simulink model "MMC_phase_hackathon_consensus_PWM_JABBAR_20260927"  (R2024b)
settings: Solver=FixedStepDiscrete  StartTime=t_init_sim  StopTime=sim_time  FixedStep=Ts  RelTol=1e-3
values from neighbouring files (symbols this model uses):
  a = 1    [script_MMC_phase_hackathon_consensus_PWM_JABBAR_20260927.m]
  C1low1_active = 1    [script_MMC_phase_hackathon_consensus_PWM_JABBAR_20260927.m]
  C2low1_active = 1    [script_MMC_phase_hackathon_consensus_PWM_JABBAR_20260927.m]
  C_bus = 4400e-6    (= 0.0044)    [script_MMC_phase_hackathon_consensus_PWM_JABBAR_20260927.m]
  C_M_extra = C_m-twist_high_side_C    [script_MMC_phase_hackathon_consensus_PWM_JABBAR_20260927.m]
  f0 = 50    [script_MMC_phase_hackathon_consensus_PWM_JABBAR_20260927.m]
  feeder_current_lower_rate_limit = -10    [script_MMC_phase_hackathon_consensus_PWM_JABBAR_20260927.m]    (also in twist_parameters.m = -500)
  feeder_current_tab = [0.328 0.217 0.162 0.132 0.109 0.094 0.083 0.075 0.068 0.062 0.058 0.054 ... (42 elements, 14x3)]    [feeder_current.mat]
  feeder_current_upper_rate_limit = 0.386/(20e-3)    (= 19.3)    [twist_parameters.m]
  is6VExternallySupplied = true    [script_MMC_phase_hackathon_consensus_PWM_JABBAR_20260927.m]
  isFeederJumperOpen = true    [script_MMC_phase_hackathon_consensus_PWM_JABBAR_20260927.m]
  L_arm = 100e-3    (= 0.1)    [script_MMC_phase_hackathon_consensus_PWM_JABBAR_20260927.m]
  m = 1    [script_MMC_phase_hackathon_consensus_PWM_JABBAR_20260927.m]
  power_losses = false    [script_MMC_phase_hackathon_consensus_PWM_JABBAR_20260927.m]
  R = 30    [script_MMC_phase_hackathon_consensus_PWM_JABBAR_20260927.m]
  R_arm = 0.2    [script_MMC_phase_hackathon_consensus_PWM_JABBAR_20260927.m]
  source_V = 0    [script_MMC_phase_hackathon_consensus_PWM_JABBAR_20260927.m]
  time_charge = 0.1    [script_MMC_phase_hackathon_consensus_PWM_JABBAR_20260927.m]
  time_decharge = 1.5    [script_MMC_phase_hackathon_consensus_PWM_JABBAR_20260927.m]
  Ts = 5e-7    (= 5e-07)    [script_MMC_phase_hackathon_consensus_PWM_JABBAR_20260927.m]
  twist_data_acquisition_delay = 50e-9    (= 5e-08)    [script_MMC_phase_hackathon_consensus_PWM_JABBAR_20260927.m]    (also in twist_parameters.m)
  twist_data_sampling_period = 1/twist_freq_data_sampling    (= 5e-05)    [script_MMC_phase_hackathon_consensus_PWM_JABBAR_20260927.m]    (also in twist_parameters.m)
  twist_dead_time = 200e-9    (= 2e-07)    [twist_parameters.m]
  twist_freq_switching = 200e3    (= 200000)    [twist_parameters.m]
  twist_high_side_adc_R = 1/(1/2e6 + 1/2e6 + 1/(330e3+5.6e3))    (= 251272.836178)    [twist_parameters.m]
  twist_high_side_C = 33e-6*4 + 4.7e-6*12    (= 0.0001884)    [twist_parameters.m]
  twist_high_side_feeder_R = 47e3+4.7e3    (= 51700)    [twist_parameters.m]
  twist_high_side_rC = 0.1    [twist_parameters.m]
  twist_low_side_adc_R = 150e3+470    (= 150470)    [twist_parameters.m]
  twist_low_side_C_ceramic = 3*4.7e-6    (= 1.41e-05)    [twist_parameters.m]
  twist_low_side_C_electrolytic = 47e-6    (= 4.7e-05)    [twist_parameters.m]
  twist_low_side_L = 33e-6    (= 3.3e-05)    [twist_parameters.m]
  twist_low_side_rC = 700e-3    (= 0.7)    [twist_parameters.m]
  twist_low_side_rL = 20e-3    (= 0.02)    [twist_parameters.m]
  twist_R_VCC = (tau_VCC/twist_high_side_C  - twist_high_side_rC)/(1-(tau_VCC/twist_high_side_C - twist_high_side_rC)/R_parallel)    (= 1110.74997822)    [twist_parameters.m]
  VDC = 48    [script_MMC_phase_hackathon_consensus_PWM_JABBAR_20260927.m]
undefined symbols (not defined in the file or in its folder): C_SM, feeder_current, gcbh, sps_rtmsupport, twist_low_side_lC
libraries: spsSeriesRLCBranchLib x135, spsTriangleGeneratorLib x60, spsMosfetLib x60, spsCurrentMeasurementLib x43, spsVoltageMeasurementLib x35, spsControlledCurrentSourceLib x30, spsDiodeLib x22, spsIdealSwitchLib x20, spsControlledVoltageSourceLib x1, spsGroundLib x1, spspowerguiLib x1
(part 8 of 19)

== system MMC_phase_hackathon_consensus_PWM_JABBAR_20260927/ /Subsystem/Subsystem1/Hardware M3/Feeder block ==
  note: Note:
      | Feeder chracteristics changed to consider threshold voltages (Vth_start = 9.7 V and Vth_stop = 8.9 V).
      | -When started, its VIN PIN consums the current generated by the lookup table fed with consumption experimental data from OwnTech.
      | -When stopped, its VIN PIN no longer consums current but its VCC PIN is modelled as a resistance calculated to match experimental results.
      | -When externally supply the 6 V used by the board, the feeder consums a constant 11.2 mA current when above threshold voltage, which is its correspondent to the minimum current in datasheet (15 mA).
  duty_cycle : Inport
  vHMeas : Inport  Port=2
  2-D Lookup Table : Lookup_n-D  Commented=on  LookupTableObject=feeder_current_tab  BreakpointsSpecification=Even spacing  BreakpointsForDimension1=[1:4]  BreakpointsForDimension2=[1:3]  BreakpointsForDimension1FirstPoint=feeder_VHigh_min  BreakpointsForDimension2FirstPoint=feeder_duty_min  BreakpointsForDimension1Spacing=feeder_VHigh_spacing  BreakpointsForDimension2Spacing=feeder_duty_spacing  TableSource=Input port  Table=feeder_current  InternalRulePriority=Speed  RndMeth=Simplest
      settings: InputPortMap=u0,u1,p221
  Constant11 : Constant  Commented=on  Value=is6VExternallySupplied
  Constant12 : Constant  Commented=on  Value=isFeederJumperOpen
  Constant2 : Constant  Commented=on  Value=0
  Constant4 : Constant  Commented=on  Value=0
  Constant5 : Constant  Commented=on
  Constant6 : Constant  Commented=on  Value=0
  Constant7 : Constant  Commented=on  Value=feeder_current_tab
  GreaterThan : RelationalOperator  Commented=on  Operator=>  OutDataTypeStr=boolean  RndMeth=Simplest  InputSameDT=off
  MATLAB Function : MATLAB Function  Commented=on  TreatAsAtomicUnit=on
  Memory : Memory  Commented=on  InheritSampleTime=on  LinearizeAsDelay=on
  Rate Limiter : RateLimiter  Commented=on  RisingSlewLimit=feeder_current_upper_rate_limit  FallingSlewLimit=feeder_current_lower_rate_limit  SampleTimeMode=inherited
  Switch : Switch  Commented=on  Criteria=u2 > Threshold  Threshold=2.05  SaturateOnIntegerOverflow=off  InputSameDT=off
  Switch10 : Switch  Commented=on  Criteria=u2 > Threshold  SaturateOnIntegerOverflow=off  InputSameDT=off
  Switch11 : Switch  Commented=on  Criteria=u2 > Threshold  SaturateOnIntegerOverflow=off  InputSameDT=off
  Switch9 : Switch  Commented=on  Criteria=u2 > Threshold  SaturateOnIntegerOverflow=off  InputSameDT=off
  Qjumper : Outport
  feeder_current : Outport  Port=2
  QVCC : Outport  Port=3
  wires:
  GreaterThan/1 -> Memory/1
  Constant2/1 -> GreaterThan/2
  Constant5/1 -> Switch11/3
  MATLAB Function/1(y) -> GreaterThan/1, Rate Limiter/1
  Constant4/1 -> Switch/3
  Switch/1 -> QVCC/1
  Switch10/1 -> Switch/1
  Memory/1 -> MATLAB Function/4(active_1)
  Constant6/1 -> Switch11/1, Switch10/1, Switch9/1
  Constant12/1 -> Switch11/2, Switch9/2, Switch10/2
  Constant11/1 -> MATLAB Function/3(isfeederdisabled)
  2-D Lookup Table/1 -> MATLAB Function/1(i_feeder)
  Rate Limiter/1 -> Switch9/3
  MATLAB Function/2(Q_VCC) -> Switch10/3
  Switch9/1 -> feeder_current/1
  Constant7/1 -> 2-D Lookup Table/3
  duty_cycle/1 -> 2-D Lookup Table/2
  vHMeas/1 -> MATLAB Function/2(vC), Switch/2, 2-D Lookup Table/1
  Switch11/1 -> Qjumper/1

== system MMC_phase_hackathon_consensus_PWM_JABBAR_20260927/ /Subsystem/Subsystem1/Hardware M3/HRTimA_1 ==
  note: PWM Timer Model
  note: Note 2:
      | All sampling times inferior than Ts = 1e-6 were desactivated or changed to Ts to reduce simulation duration
  note: Note 3:
      | PWM generator original resolution value at 100 ns
  note: Note 1:
      | HRTim modified adding block mode, equivalent to shield.power.stop(ALL);
  Duty cycle input : Inport
  Block : Inport  Port=2
  Constant : Constant  Value=0
  Dead Time : TransportDelay  Commented=on  DelayTime=twist_dead_time
  Demux : Demux  Outputs=2
  Logical Operator : Logic  AllPortsSameDT=off  OutDataTypeStr=boolean
  PWM Generator (2-Level) : Subsystem  AncestorBlock=|  DialogController=POWERSYS.PowerSysDialog  LoadFcn=sps_rtmsupport('LoadFcn', gcbh);  StartFcn=sps_rtmsupport('StartFcn', gcbh);  StopFcn=sps_rtmsupport('StopFcn', gcbh);  BlockChoice=InternalUref  mask(PWM Generator (2-Level)){ModulatorType=Single-phase half-bridge (2 pulses), ModulatorMode=Unsynchronized, Fc=twist_freq_switching, Pc=144, nF=27, MinMax=[0 1], SamplingTechnique=Symmetrical regular (single edge), ModulatingSignals=off, m=0.8, Freq=60, Phase=0, Ts=Ts, ShowCarrierOutport=off}
      | spsPWMGenerator2LevelLib/PWM Generator
      | (2-Level)
      mask prompts: ModulatorType "Generator type:"; ModulatorMode "Mode of operation:"; Fc "Frequency (Hz):"; Pc "Initial phase (degrees):"; nF "Switching ratio (carrier frequency / output frequency):"; MinMax "Minimum and maximum values: [ Min  Max ]"; SamplingTechnique "Sampling technique:"; ModulatingSignals "Internal generation of reference signal"; m "Modulation index:"; Freq "Frequency (Hz):"; Phase "Phase (degrees):"; Ts "Sample time (s):"; ShowCarrierOutport "Show measurement port"
      mask help:
      | Generate pulses for PWM-controlled 2-Level converter, using carrier-based two-level PWM method. The block can control switching devices of single-phase half-bridge, single-phase full-bridge (unipolar or bipolar modulation) or three-phase bridge.
      |
      | When the Synchronized mode of operation is selected, a second input is added to the block, and the internal generation of modulating signal is disabled. Use input 2 (wt) to synchronize the carrier.
      mask init:
      | sps = powericon('PWMGenerator2LevelInit',gcb,ModulatorType,SamplingTechnique,ModulatorMode,nF,Fc,MinMax,Pc,ShowCarrierOutport,ModulatingSignals,m,Freq,Phase,Ts);
      settings: CopyFcn=sps_rtmsupport('CopyFcn', gcbh);  DeleteFcn=sps_rtmsupport('DeleteFcn', gcbh);  UndoDeleteFcn=sps_rtmsupport('UndoDeleteFcn', gcbh);  ModelCloseFcn=sps_rtmsupport('ModelCloseFcn', gcbh);  PreSaveFcn=sps_rtmsupport('PreSaveFcn', gcbh);  PostSaveFcn=sps_rtmsupport('PostSaveFcn', gcbh);  NameChangeFcn=sps_rtmsupport('NameChangeFcn', gcbh);  PreCopyFcn=sps_rtmsupport('PreCopyFcn', gcbh);  OpenFcn="sps_rtmsupport('OpenFcn', gcbh, [1   2   7   8  13]);"  CloseFcn=sps_rtmsupport('CloseFcn', gcbh);  PreDeleteFcn=sps_rtmsupport('PreDeleteFcn', gcbh);
      mask Help: helpview(psbhelp);
      mask TypeOptions ModulatorType: Single-phase half-bridge (2 pulses) | Single-phase full-bridge (4 pulses) | Single-phase full-bridge - Bipolar modulation (4 pulses) | Three-phase bridge (6 pulses)
      mask TypeOptions ModulatorMode: Synchronized | Unsynchronized
      mask Callback ModulatorMode: powericon('PWMGenerator2LevelCback',gcb);
      mask TypeOptions SamplingTechnique: Natural | Asymmetrical regular (double edge) | Symmetrical regular (single edge)
      mask Callback ModulatingSignals: powericon('PWMGenerator2LevelCback',gcb);
      mask DialogControl Container3 Prompt: Carrier
      mask DialogControl ModulatingSignalParameters Prompt: Reference signal
  Peak acq : ZeroOrderHold  Commented=on  SampleTime=twist_data_acquisition_delay
  Switch : Switch  Criteria=u2 > Threshold  SaturateOnIntegerOverflow=off  InputSameDT=off
  Switch1 : Switch  Criteria=u2 > Threshold  SaturateOnIntegerOverflow=off  InputSameDT=off
  High-Side Q : Outport
  Low-Side Q : Outport  Port=2
  Carry Leg : Outport  Port=3
  wires:
  Demux/1 -> Switch/3  "high side"
  Duty cycle input/1 -> PWM Generator (2-Level)/1(Uref)  "duty_cycle"
  PWM Generator (2-Level)/2(Carry) -> Carry Leg/1, Peak acq/1  "carrier"
  Block/1 -> Switch/2, Switch1/2  "block"
  Demux/2 -> Switch1/3  "low side"
  Switch1/1 -> Low-Side Q/1
  Switch/1 -> High-Side Q/1
  Constant/1 -> Switch1/1, Switch/1
  PWM Generator (2-Level)/1(P) -> Demux/1, Dead Time/1, Logical Operator/1, Logical Operator/2  "PWM_out"

== system MMC_phase_hackathon_consensus_PWM_JABBAR_20260927/ /Subsystem/Subsystem1/Hardware M3/HRTimA_2 ==
  note: PWM Timer Model
  note: Note 2:
      | All sampling times inferior than Ts = 1e-6 were desactivated or changed to Ts to reduce simulation duration
  note: Note 3:
      | PWM generator original resolution value at 100 ns
  note: Note 1:
      | HRTim modified adding block mode, equivalent to shield.power.stop(ALL);
  Duty cycle input : Inport
  Block : Inport  Port=2
  Constant : Constant  Value=0
  Dead Time : TransportDelay  Commented=on  DelayTime=twist_dead_time
  Demux : Demux  Outputs=2
  Logical Operator : Logic  AllPortsSameDT=off  OutDataTypeStr=boolean
  PWM Generator (2-Level) : Subsystem  AncestorBlock=|  DialogController=POWERSYS.PowerSysDialog  LoadFcn=sps_rtmsupport('LoadFcn', gcbh);  StartFcn=sps_rtmsupport('StartFcn', gcbh);  StopFcn=sps_rtmsupport('StopFcn', gcbh);  BlockChoice=InternalUref  mask(PWM Generator (2-Level)){ModulatorType=Single-phase half-bridge (2 pulses), ModulatorMode=Unsynchronized, Fc=twist_freq_switching, Pc=0, nF=27, MinMax=[0 1], SamplingTechnique=Symmetrical regular (single edge), ModulatingSignals=off, m=0.8, Freq=60, Phase=0, Ts=Ts, ShowCarrierOutport=off}
      | spsPWMGenerator2LevelLib/PWM Generator
      | (2-Level)
      mask prompts: ModulatorType "Generator type:"; ModulatorMode "Mode of operation:"; Fc "Frequency (Hz):"; Pc "Initial phase (degrees):"; nF "Switching ratio (carrier frequency / output frequency):"; MinMax "Minimum and maximum values: [ Min  Max ]"; SamplingTechnique "Sampling technique:"; ModulatingSignals "Internal generation of reference signal"; m "Modulation index:"; Freq "Frequency (Hz):"; Phase "Phase (degrees):"; Ts "Sample time (s):"; ShowCarrierOutport "Show measurement port"
      mask help:
      | Generate pulses for PWM-controlled 2-Level converter, using carrier-based two-level PWM method. The block can control switching devices of single-phase half-bridge, single-phase full-bridge (unipolar or bipolar modulation) or three-phase bridge.
      |
      | When the Synchronized mode of operation is selected, a second input is added to the block, and the internal generation of modulating signal is disabled. Use input 2 (wt) to synchronize the carrier.
      mask init:
      | sps = powericon('PWMGenerator2LevelInit',gcb,ModulatorType,SamplingTechnique,ModulatorMode,nF,Fc,MinMax,Pc,ShowCarrierOutport,ModulatingSignals,m,Freq,Phase,Ts);
      settings: CopyFcn=sps_rtmsupport('CopyFcn', gcbh);  DeleteFcn=sps_rtmsupport('DeleteFcn', gcbh);  UndoDeleteFcn=sps_rtmsupport('UndoDeleteFcn', gcbh);  ModelCloseFcn=sps_rtmsupport('ModelCloseFcn', gcbh);  PreSaveFcn=sps_rtmsupport('PreSaveFcn', gcbh);  PostSaveFcn=sps_rtmsupport('PostSaveFcn', gcbh);  NameChangeFcn=sps_rtmsupport('NameChangeFcn', gcbh);  PreCopyFcn=sps_rtmsupport('PreCopyFcn', gcbh);  OpenFcn="sps_rtmsupport('OpenFcn', gcbh, [1   2   7   8  13]);"  CloseFcn=sps_rtmsupport('CloseFcn', gcbh);  PreDeleteFcn=sps_rtmsupport('PreDeleteFcn', gcbh);
      mask Help: helpview(psbhelp);
      mask TypeOptions ModulatorType: Single-phase half-bridge (2 pulses) | Single-phase full-bridge (4 pulses) | Single-phase full-bridge - Bipolar modulation (4 pulses) | Three-phase bridge (6 pulses)
      mask TypeOptions ModulatorMode: Synchronized | Unsynchronized
      mask Callback ModulatorMode: powericon('PWMGenerator2LevelCback',gcb);
      mask TypeOptions SamplingTechnique: Natural | Asymmetrical regular (double edge) | Symmetrical regular (single edge)
      mask Callback ModulatingSignals: powericon('PWMGenerator2LevelCback',gcb);
      mask DialogControl Container3 Prompt: Carrier
      mask DialogControl ModulatingSignalParameters Prompt: Reference signal
  Peak acq : ZeroOrderHold  Commented=on  SampleTime=twist_data_acquisition_delay
  Switch : Switch  Criteria=u2 > Threshold  SaturateOnIntegerOverflow=off  InputSameDT=off
  Switch1 : Switch  Criteria=u2 > Threshold  SaturateOnIntegerOverflow=off  InputSameDT=off
  High-Side Q : Outport
  Low-Side Q : Outport  Port=2
  Carry Leg : Outport  Port=3
  wires:
  Logical Operator/1 -> Demux/1
  Demux/1 -> Switch/3  "high side"
  Duty cycle input/1 -> PWM Generator (2-Level)/1(Uref)  "duty_cycle"
  PWM Generator (2-Level)/2(Carry) -> Carry Leg/1, Peak acq/1  "carrier"
  Block/1 -> Switch/2, Switch1/2  "block"
  Demux/2 -> Switch1/3  "low side"
  Switch1/1 -> Low-Side Q/1
  Switch/1 -> High-Side Q/1
  Constant/1 -> Switch1/1, Switch/1
  PWM Generator (2-Level)/1(P) -> Dead Time/1, Logical Operator/1, Logical Operator/2  "PWM_out"

== system MMC_phase_hackathon_consensus_PWM_JABBAR_20260927/ /Subsystem/Subsystem1/Hardware M3/Measurement block ==
  note: Note:
      | All sampling times inferior than Ts = 1e-6 were desactivated or changed to Ts to reduce simulation duration
  i1Meas : Inport
  vHMeas : Inport  Port=2
  v1Meas : Inport  Port=3
  i2Meas : Inport  Port=4
  v2Meas : Inport  Port=5
  iHMeas : Inport  Port=6
  Carry_leg_1 : Inport  Port=7
  Gain : Gain  Gain=-1
  Zero-Order Hold{1..6} (6 alike) : ZeroOrderHold  Commented=on  SampleTime=twist_data_sampling_period
  i1Low acquisition : Subsystem  Commented=on
  i2Low acquisition : Subsystem  Commented=on
  iHigh acquisition : Subsystem  Commented=on
  v1Low acquisition : Subsystem  Commented=on
  v2Low acquisition : Subsystem  Commented=on
  vHigh acquisition : Subsystem  Commented=on
  i1 : Outport
  i2 : Outport  Port=2
  v1 : Outport  Port=3
  v2 : Outport  Port=4
  vH : Outport  Port=5
  iH : Outport  Port=6
  wires:
  Carry_leg_1/1 -> v2Low acquisition/2(In2), iHigh acquisition/2(In2), i2Low acquisition/2(In2), vHigh acquisition/2(In2), v1Low acquisition/2(In2), i1Low acquisition/2(In2)
  v2Low acquisition/1(v2Meas) -> Zero-Order Hold5/1
  v1Meas/1 -> v1/1, v1Low acquisition/1(In1)
  i2Low acquisition/1(i2Meas) -> Zero-Order Hold4/1
  vHigh acquisition/1(vHMeas) -> Zero-Order Hold2/1
  v1Low acquisition/1(v1Meas) -> Zero-Order Hold3/1
  vHMeas/1 -> vH/1, vHigh acquisition/1(In1)
  i2Meas/1 -> i2/1, i2Low acquisition/1(In1)
  iHigh acquisition/1(iHMeas) -> Zero-Order Hold6/1
  v2Meas/1 -> v2/1, v2Low acquisition/1(In1)
  iHMeas/1 -> iH/1, iHigh acquisition/1(In1)
  i1Low acquisition/1(i1Meas) -> Zero-Order Hold1/1
  i1Meas/1 -> Gain/1, i1Low acquisition/1(In1)
  Gain/1 -> i1/1

== system MMC_phase_hackathon_consensus_PWM_JABBAR_20260927/ /Subsystem/Subsystem1/Hardware M3/Power losses branch 1 ==
  note: Output signals
  note: Input signals
  note: Power losses calculations
  note: Note:
      | Power losses are modelled but not used in this specific simulation since they are small for a MMC module (low switching frequency).
      |
      | This power losses estimation can't be used when High voltage is 0.
  VHigh : Inport
  ILow : Inport  Port=2
  VLow : Inport  Port=3
  Add : Sum  Commented=on  Inputs=++++
  Branch DT loss : MATLAB Function  Commented=on  TreatAsAtomicUnit=on
  Branch cond loss : MATLAB Function  Commented=on  TreatAsAtomicUnit=on
  Branch gate loss : MATLAB Function  Commented=on  TreatAsAtomicUnit=on
  Branch switching loss : MATLAB Function  Commented=on  TreatAsAtomicUnit=on
  Divide1 : Product  Commented=on  Inputs=/*
  From : From  Commented=on  GotoTag=VHigh
  From1 : From  Commented=on  GotoTag=VLow
  From2 : From  Commented=on  GotoTag=ILow
  Goto3 : Goto  Commented=on  GotoTag=ILoss
  i1Loss : Outport
  wires:
  Branch switching loss/1(twist_FET_Psw) -> Add/2
  From2/1 -> Branch switching loss/2(ILow), Branch cond loss/3(ILow), Branch DT loss/1(ILow)
  Branch gate loss/1(twist_FET_Pg) -> Add/1
  Branch cond loss/1(twist_FET_Pcond) -> Add/4
  From/1 -> Divide1/1, Branch cond loss/1(VHigh), Branch switching loss/1(VHigh)
  Branch DT loss/1(twist_FET_Pdt) -> Add/3
  From1/1 -> Branch cond loss/2(VLow)
  Divide1/1 -> Goto3/1  "i1Loss"
  VHigh/1 -> [VHigh]
  ILow/1 -> [ILow]
  VLow/1 -> [VLow]
  [ILoss] -> i1Loss/1
  Add/1 -> Divide1/2

== system MMC_phase_hackathon_consensus_PWM_JABBAR_20260927/ /Subsystem/Subsystem1/Hardware M3/Power losses branch 2 ==
  note: Output signals
  note: Input signals
  note: Power losses calculations
  note: Note:
      | Power losses are modelled but not used in this specific simulation since they are small for a MMC module (low switching frequency).
      |
      | This power losses estimation can't be used when High voltage is 0.
  VHigh : Inport
  ILow : Inport  Port=2
  VLow : Inport  Port=3
  Add : Sum  Commented=on  Inputs=++++
  Branch DT loss : MATLAB Function  Commented=on  TreatAsAtomicUnit=on
  Branch cond loss : MATLAB Function  Commented=on  TreatAsAtomicUnit=on
  Branch gate loss : MATLAB Function  Commented=on  TreatAsAtomicUnit=on
  Branch switching loss : MATLAB Function  Commented=on  TreatAsAtomicUnit=on
  Divide1 : Product  Commented=on  Inputs=/*
  From : From  Commented=on  GotoTag=VHigh
  From1 : From  Commented=on  GotoTag=VLow
  From2 : From  Commented=on  GotoTag=ILow
  Goto3 : Goto  Commented=on  GotoTag=ILoss
  i1Loss : Outport
  wires:
  Branch switching loss/1(twist_FET_Psw) -> Add/2
  From2/1 -> Branch switching loss/2(ILow), Branch cond loss/3(ILow), Branch DT loss/1(ILow)
  Branch gate loss/1(twist_FET_Pg) -> Add/1
  Branch cond loss/1(twist_FET_Pcond) -> Add/4
  From/1 -> Divide1/1, Branch cond loss/1(VHigh), Branch switching loss/1(VHigh)
  Branch DT loss/1(twist_FET_Pdt) -> Add/3
  From1/1 -> Branch cond loss/2(VLow)
  Divide1/1 -> Goto3/1  "i1Loss"
  VHigh/1 -> [VHigh]
  ILow/1 -> [ILow]
  VLow/1 -> [VLow]
  [ILoss] -> i1Loss/1
  Add/1 -> Divide1/2

== system MMC_phase_hackathon_consensus_PWM_JABBAR_20260927/ /Subsystem/Subsystem1/Hardware M4/Driver block 1 ==
  command_Q1 : Inport
  command_Q2 : Inport  Port=2
  Q1 : Outport
  Q2 : Outport  Port=2
  wires:
  command_Q1/1 -> Q1/1
  command_Q2/1 -> Q2/1

== system MMC_phase_hackathon_consensus_PWM_JABBAR_20260927/ /Subsystem/Subsystem1/Hardware M4/Driver block 2 ==
  command_Q3 : Inport
  command_Q4 : Inport  Port=2
  Q3 : Outport
  Q4 : Outport  Port=2
  wires:
  command_Q3/1 -> Q3/1
  command_Q4/1 -> Q4/1

== system MMC_phase_hackathon_consensus_PWM_JABBAR_20260927/ /Subsystem/Subsystem1/Hardware M4/Feeder block ==
  note: Note:
      | Feeder chracteristics changed to consider threshold voltages (Vth_start = 9.7 V and Vth_stop = 8.9 V).
      | -When started, its VIN PIN consums the current generated by the lookup table fed with consumption experimental data from OwnTech.
      | -When stopped, its VIN PIN no longer consums current but its VCC PIN is modelled as a resistance calculated to match experimental results.
      | -When externally supply the 6 V used by the board, the feeder consums a constant 11.2 mA current when above threshold voltage, which is its correspondent to the minimum current in datasheet (15 mA).
  duty_cycle : Inport
  vHMeas : Inport  Port=2
  2-D Lookup Table : Lookup_n-D  Commented=on  LookupTableObject=feeder_current_tab  BreakpointsSpecification=Even spacing  BreakpointsForDimension1=[1:4]  BreakpointsForDimension2=[1:3]  BreakpointsForDimension1FirstPoint=feeder_VHigh_min  BreakpointsForDimension2FirstPoint=feeder_duty_min  BreakpointsForDimension1Spacing=feeder_VHigh_spacing  BreakpointsForDimension2Spacing=feeder_duty_spacing  TableSource=Input port  Table=feeder_current  InternalRulePriority=Speed  RndMeth=Simplest
      settings: InputPortMap=u0,u1,p221
  Constant11 : Constant  Commented=on  Value=is6VExternallySupplied
  Constant12 : Constant  Commented=on  Value=isFeederJumperOpen
  Constant2 : Constant  Commented=on  Value=0
  Constant4 : Constant  Commented=on  Value=0
  Constant5 : Constant  Commented=on
  Constant6 : Constant  Commented=on  Value=0
  Constant7 : Constant  Commented=on  Value=feeder_current_tab
  GreaterThan : RelationalOperator  Commented=on  Operator=>  OutDataTypeStr=boolean  RndMeth=Simplest  InputSameDT=off
  MATLAB Function : MATLAB Function  Commented=on  TreatAsAtomicUnit=on
  Memory : Memory  Commented=on  InheritSampleTime=on  LinearizeAsDelay=on
  Rate Limiter : RateLimiter  Commented=on  RisingSlewLimit=feeder_current_upper_rate_limit  FallingSlewLimit=feeder_current_lower_rate_limit  SampleTimeMode=inherited
  Switch : Switch  Commented=on  Criteria=u2 > Threshold  Threshold=2.05  SaturateOnIntegerOverflow=off  InputSameDT=off
  Switch10 : Switch  Commented=on  Criteria=u2 > Threshold  SaturateOnIntegerOverflow=off  InputSameDT=off
  Switch11 : Switch  Commented=on  Criteria=u2 > Threshold  SaturateOnIntegerOverflow=off  InputSameDT=off
  Switch9 : Switch  Commented=on  Criteria=u2 > Threshold  SaturateOnIntegerOverflow=off  InputSameDT=off
  Qjumper : Outport
  feeder_current : Outport  Port=2
  QVCC : Outport  Port=3
  wires:
  GreaterThan/1 -> Memory/1
  Constant2/1 -> GreaterThan/2
  Constant5/1 -> Switch11/3
  MATLAB Function/1(y) -> GreaterThan/1, Rate Limiter/1
  Constant4/1 -> Switch/3
  Switch/1 -> QVCC/1
  Switch10/1 -> Switch/1
  Memory/1 -> MATLAB Function/4(active_1)
  Constant6/1 -> Switch11/1, Switch10/1, Switch9/1
  Constant12/1 -> Switch11/2, Switch9/2, Switch10/2
  Constant11/1 -> MATLAB Function/3(isfeederdisabled)
  2-D Lookup Table/1 -> MATLAB Function/1(i_feeder)
  Rate Limiter/1 -> Switch9/3
  MATLAB Function/2(Q_VCC) -> Switch10/3
  Switch9/1 -> feeder_current/1
  Constant7/1 -> 2-D Lookup Table/3
  duty_cycle/1 -> 2-D Lookup Table/2
  vHMeas/1 -> MATLAB Function/2(vC), Switch/2, 2-D Lookup Table/1
  Switch11/1 -> Qjumper/1

== system MMC_phase_hackathon_consensus_PWM_JABBAR_20260927/ /Subsystem/Subsystem1/Hardware M4/HRTimA_1 ==
  note: PWM Timer Model
  note: Note 2:
      | All sampling times inferior than Ts = 1e-6 were desactivated or changed to Ts to reduce simulation duration
  note: Note 3:
      | PWM generator original resolution value at 100 ns
  note: Note 1:
      | HRTim modified adding block mode, equivalent to shield.power.stop(ALL);
  Duty cycle input : Inport
  Block : Inport  Port=2
  Constant : Constant  Value=0
  Dead Time : TransportDelay  Commented=on  DelayTime=twist_dead_time
  Demux : Demux  Outputs=2
  Logical Operator : Logic  AllPortsSameDT=off  OutDataTypeStr=boolean
  PWM Generator (2-Level) : Subsystem  AncestorBlock=|  DialogController=POWERSYS.PowerSysDialog  LoadFcn=sps_rtmsupport('LoadFcn', gcbh);  StartFcn=sps_rtmsupport('StartFcn', gcbh);  StopFcn=sps_rtmsupport('StopFcn', gcbh);  BlockChoice=InternalUref  mask(PWM Generator (2-Level)){ModulatorType=Single-phase half-bridge (2 pulses), ModulatorMode=Unsynchronized, Fc=twist_freq_switching, Pc=216, nF=27, MinMax=[0 1], SamplingTechnique=Symmetrical regular (single edge), ModulatingSignals=off, m=0.8, Freq=60, Phase=0, Ts=Ts, ShowCarrierOutport=off}
      | spsPWMGenerator2LevelLib/PWM Generator
      | (2-Level)
      mask prompts: ModulatorType "Generator type:"; ModulatorMode "Mode of operation:"; Fc "Frequency (Hz):"; Pc "Initial phase (degrees):"; nF "Switching ratio (carrier frequency / output frequency):"; MinMax "Minimum and maximum values: [ Min  Max ]"; SamplingTechnique "Sampling technique:"; ModulatingSignals "Internal generation of reference signal"; m "Modulation index:"; Freq "Frequency (Hz):"; Phase "Phase (degrees):"; Ts "Sample time (s):"; ShowCarrierOutport "Show measurement port"
      mask help:
      | Generate pulses for PWM-controlled 2-Level converter, using carrier-based two-level PWM method. The block can control switching devices of single-phase half-bridge, single-phase full-bridge (unipolar or bipolar modulation) or three-phase bridge.
      |
      | When the Synchronized mode of operation is selected, a second input is added to the block, and the internal generation of modulating signal is disabled. Use input 2 (wt) to synchronize the carrier.
      mask init:
      | sps = powericon('PWMGenerator2LevelInit',gcb,ModulatorType,SamplingTechnique,ModulatorMode,nF,Fc,MinMax,Pc,ShowCarrierOutport,ModulatingSignals,m,Freq,Phase,Ts);
      settings: CopyFcn=sps_rtmsupport('CopyFcn', gcbh);  DeleteFcn=sps_rtmsupport('DeleteFcn', gcbh);  UndoDeleteFcn=sps_rtmsupport('UndoDeleteFcn', gcbh);  ModelCloseFcn=sps_rtmsupport('ModelCloseFcn', gcbh);  PreSaveFcn=sps_rtmsupport('PreSaveFcn', gcbh);  PostSaveFcn=sps_rtmsupport('PostSaveFcn', gcbh);  NameChangeFcn=sps_rtmsupport('NameChangeFcn', gcbh);  PreCopyFcn=sps_rtmsupport('PreCopyFcn', gcbh);  OpenFcn="sps_rtmsupport('OpenFcn', gcbh, [1   2   7   8  13]);"  CloseFcn=sps_rtmsupport('CloseFcn', gcbh);  PreDeleteFcn=sps_rtmsupport('PreDeleteFcn', gcbh);
      mask Help: helpview(psbhelp);
      mask TypeOptions ModulatorType: Single-phase half-bridge (2 pulses) | Single-phase full-bridge (4 pulses) | Single-phase full-bridge - Bipolar modulation (4 pulses) | Three-phase bridge (6 pulses)
      mask TypeOptions ModulatorMode: Synchronized | Unsynchronized
      mask Callback ModulatorMode: powericon('PWMGenerator2LevelCback',gcb);
      mask TypeOptions SamplingTechnique: Natural | Asymmetrical regular (double edge) | Symmetrical regular (single edge)
      mask Callback ModulatingSignals: powericon('PWMGenerator2LevelCback',gcb);
      mask DialogControl Container3 Prompt: Carrier
      mask DialogControl ModulatingSignalParameters Prompt: Reference signal
  Peak acq : ZeroOrderHold  Commented=on  SampleTime=twist_data_acquisition_delay
  Switch : Switch  Criteria=u2 > Threshold  SaturateOnIntegerOverflow=off  InputSameDT=off
  Switch1 : Switch  Criteria=u2 > Threshold  SaturateOnIntegerOverflow=off  InputSameDT=off
  High-Side Q : Outport
  Low-Side Q : Outport  Port=2
  Carry Leg : Outport  Port=3
  wires:
  Demux/1 -> Switch/3  "high side"
  Duty cycle input/1 -> PWM Generator (2-Level)/1(Uref)  "duty_cycle"
  PWM Generator (2-Level)/2(Carry) -> Carry Leg/1, Peak acq/1  "carrier"
  Block/1 -> Switch/2, Switch1/2  "block"
  Demux/2 -> Switch1/3  "low side"
  Switch1/1 -> Low-Side Q/1
  Switch/1 -> High-Side Q/1
  Constant/1 -> Switch1/1, Switch/1
  PWM Generator (2-Level)/1(P) -> Demux/1, Dead Time/1, Logical Operator/1, Logical Operator/2  "PWM_out"

== system MMC_phase_hackathon_consensus_PWM_JABBAR_20260927/ /Subsystem/Subsystem1/Hardware M4/HRTimA_2 ==
  note: PWM Timer Model
  note: Note 2:
      | All sampling times inferior than Ts = 1e-6 were desactivated or changed to Ts to reduce simulation duration
  note: Note 3:
      | PWM generator original resolution value at 100 ns
  note: Note 1:
      | HRTim modified adding block mode, equivalent to shield.power.stop(ALL);
  Duty cycle input : Inport
  Block : Inport  Port=2
  Constant : Constant  Value=0
  Dead Time : TransportDelay  Commented=on  DelayTime=twist_dead_time
  Demux : Demux  Outputs=2
  Logical Operator : Logic  AllPortsSameDT=off  OutDataTypeStr=boolean
  PWM Generator (2-Level) : Subsystem  AncestorBlock=|  DialogController=POWERSYS.PowerSysDialog  LoadFcn=sps_rtmsupport('LoadFcn', gcbh);  StartFcn=sps_rtmsupport('StartFcn', gcbh);  StopFcn=sps_rtmsupport('StopFcn', gcbh);  BlockChoice=InternalUref  mask(PWM Generator (2-Level)){ModulatorType=Single-phase half-bridge (2 pulses), ModulatorMode=Unsynchronized, Fc=twist_freq_switching, Pc=0, nF=27, MinMax=[0 1], SamplingTechnique=Symmetrical regular (single edge), ModulatingSignals=off, m=0.8, Freq=60, Phase=0, Ts=Ts, ShowCarrierOutport=off}
      | spsPWMGenerator2LevelLib/PWM Generator
      | (2-Level)
      mask prompts: ModulatorType "Generator type:"; ModulatorMode "Mode of operation:"; Fc "Frequency (Hz):"; Pc "Initial phase (degrees):"; nF "Switching ratio (carrier frequency / output frequency):"; MinMax "Minimum and maximum values: [ Min  Max ]"; SamplingTechnique "Sampling technique:"; ModulatingSignals "Internal generation of reference signal"; m "Modulation index:"; Freq "Frequency (Hz):"; Phase "Phase (degrees):"; Ts "Sample time (s):"; ShowCarrierOutport "Show measurement port"
      mask help:
      | Generate pulses for PWM-controlled 2-Level converter, using carrier-based two-level PWM method. The block can control switching devices of single-phase half-bridge, single-phase full-bridge (unipolar or bipolar modulation) or three-phase bridge.
      |
      | When the Synchronized mode of operation is selected, a second input is added to the block, and the internal generation of modulating signal is disabled. Use input 2 (wt) to synchronize the carrier.
      mask init:
      | sps = powericon('PWMGenerator2LevelInit',gcb,ModulatorType,SamplingTechnique,ModulatorMode,nF,Fc,MinMax,Pc,ShowCarrierOutport,ModulatingSignals,m,Freq,Phase,Ts);
      settings: CopyFcn=sps_rtmsupport('CopyFcn', gcbh);  DeleteFcn=sps_rtmsupport('DeleteFcn', gcbh);  UndoDeleteFcn=sps_rtmsupport('UndoDeleteFcn', gcbh);  ModelCloseFcn=sps_rtmsupport('ModelCloseFcn', gcbh);  PreSaveFcn=sps_rtmsupport('PreSaveFcn', gcbh);  PostSaveFcn=sps_rtmsupport('PostSaveFcn', gcbh);  NameChangeFcn=sps_rtmsupport('NameChangeFcn', gcbh);  PreCopyFcn=sps_rtmsupport('PreCopyFcn', gcbh);  OpenFcn="sps_rtmsupport('OpenFcn', gcbh, [1   2   7   8  13]);"  CloseFcn=sps_rtmsupport('CloseFcn', gcbh);  PreDeleteFcn=sps_rtmsupport('PreDeleteFcn', gcbh);
      mask Help: helpview(psbhelp);
      mask TypeOptions ModulatorType: Single-phase half-bridge (2 pulses) | Single-phase full-bridge (4 pulses) | Single-phase full-bridge - Bipolar modulation (4 pulses) | Three-phase bridge (6 pulses)
      mask TypeOptions ModulatorMode: Synchronized | Unsynchronized
      mask Callback ModulatorMode: powericon('PWMGenerator2LevelCback',gcb);
      mask TypeOptions SamplingTechnique: Natural | Asymmetrical regular (double edge) | Symmetrical regular (single edge)
      mask Callback ModulatingSignals: powericon('PWMGenerator2LevelCback',gcb);
      mask DialogControl Container3 Prompt: Carrier
      mask DialogControl ModulatingSignalParameters Prompt: Reference signal
  Peak acq : ZeroOrderHold  Commented=on  SampleTime=twist_data_acquisition_delay
  Switch : Switch  Criteria=u2 > Threshold  SaturateOnIntegerOverflow=off  InputSameDT=off
  Switch1 : Switch  Criteria=u2 > Threshold  SaturateOnIntegerOverflow=off  InputSameDT=off
  High-Side Q : Outport
  Low-Side Q : Outport  Port=2
  Carry Leg : Outport  Port=3
  wires:
  Logical Operator/1 -> Demux/1
  Demux/1 -> Switch/3  "high side"
  Duty cycle input/1 -> PWM Generator (2-Level)/1(Uref)  "duty_cycle"
  PWM Generator (2-Level)/2(Carry) -> Carry Leg/1, Peak acq/1  "carrier"
  Block/1 -> Switch/2, Switch1/2  "block"
  Demux/2 -> Switch1/3  "low side"
  Switch1/1 -> Low-Side Q/1
  Switch/1 -> High-Side Q/1
  Constant/1 -> Switch1/1, Switch/1
  PWM Generator (2-Level)/1(P) -> Dead Time/1, Logical Operator/1, Logical Operator/2  "PWM_out"

== system MMC_phase_hackathon_consensus_PWM_JABBAR_20260927/ /Subsystem/Subsystem1/Hardware M4/Measurement block ==
  note: Note:
      | All sampling times inferior than Ts = 1e-6 were desactivated or changed to Ts to reduce simulation duration
  i1Meas : Inport
  vHMeas : Inport  Port=2
  v1Meas : Inport  Port=3
  i2Meas : Inport  Port=4
  v2Meas : Inport  Port=5
  iHMeas : Inport  Port=6
  Carry_leg_1 : Inport  Port=7
  Gain : Gain  Gain=-1
  Zero-Order Hold{1..6} (6 alike) : ZeroOrderHold  Commented=on  SampleTime=twist_data_sampling_period
  i1Low acquisition : Subsystem  Commented=on
  i2Low acquisition : Subsystem  Commented=on
  iHigh acquisition : Subsystem  Commented=on
  v1Low acquisition : Subsystem  Commented=on
  v2Low acquisition : Subsystem  Commented=on
  vHigh acquisition : Subsystem  Commented=on
  i1 : Outport
  i2 : Outport  Port=2
  v1 : Outport  Port=3
  v2 : Outport  Port=4
  vH : Outport  Port=5
  iH : Outport  Port=6
  wires:
  Carry_leg_1/1 -> v2Low acquisition/2(In2), iHigh acquisition/2(In2), i2Low acquisition/2(In2), vHigh acquisition/2(In2), v1Low acquisition/2(In2), i1Low acquisition/2(In2)
  v2Low acquisition/1(v2Meas) -> Zero-Order Hold5/1
  v1Meas/1 -> v1/1, v1Low acquisition/1(In1)
  i2Low acquisition/1(i2Meas) -> Zero-Order Hold4/1
  vHigh acquisition/1(vHMeas) -> Zero-Order Hold2/1
  v1Low acquisition/1(v1Meas) -> Zero-Order Hold3/1
  vHMeas/1 -> vH/1, vHigh acquisition/1(In1)
  i2Meas/1 -> i2/1, i2Low acquisition/1(In1)
  iHigh acquisition/1(iHMeas) -> Zero-Order Hold6/1
  v2Meas/1 -> v2/1, v2Low acquisition/1(In1)
  iHMeas/1 -> iH/1, iHigh acquisition/1(In1)
  i1Low acquisition/1(i1Meas) -> Zero-Order Hold1/1
  i1Meas/1 -> Gain/1, i1Low acquisition/1(In1)
  Gain/1 -> i1/1

== system MMC_phase_hackathon_consensus_PWM_JABBAR_20260927/ /Subsystem/Subsystem1/Hardware M4/Power losses branch 1 ==
  note: Output signals
  note: Input signals
  note: Power losses calculations
  note: Note:
      | Power losses are modelled but not used in this specific simulation since they are small for a MMC module (low switching frequency).
      |
      | This power losses estimation can't be used when High voltage is 0.
  VHigh : Inport
  ILow : Inport  Port=2
  VLow : Inport  Port=3
  Add : Sum  Commented=on  Inputs=++++
  Branch DT loss : MATLAB Function  Commented=on  TreatAsAtomicUnit=on
  Branch cond loss : MATLAB Function  Commented=on  TreatAsAtomicUnit=on
  Branch gate loss : MATLAB Function  Commented=on  TreatAsAtomicUnit=on
  Branch switching loss : MATLAB Function  Commented=on  TreatAsAtomicUnit=on
  Divide1 : Product  Commented=on  Inputs=/*
  From : From  Commented=on  GotoTag=VHigh
  From1 : From  Commented=on  GotoTag=VLow
  From2 : From  Commented=on  GotoTag=ILow
  Goto3 : Goto  Commented=on  GotoTag=ILoss
  i1Loss : Outport
  wires:
  Branch switching loss/1(twist_FET_Psw) -> Add/2
  From2/1 -> Branch switching loss/2(ILow), Branch cond loss/3(ILow), Branch DT loss/1(ILow)
  Branch gate loss/1(twist_FET_Pg) -> Add/1
  Branch cond loss/1(twist_FET_Pcond) -> Add/4
  From/1 -> Divide1/1, Branch cond loss/1(VHigh), Branch switching loss/1(VHigh)
  Branch DT loss/1(twist_FET_Pdt) -> Add/3
  From1/1 -> Branch cond loss/2(VLow)
  Divide1/1 -> Goto3/1  "i1Loss"
  VHigh/1 -> [VHigh]
  ILow/1 -> [ILow]
  VLow/1 -> [VLow]
  [ILoss] -> i1Loss/1
  Add/1 -> Divide1/2

== system MMC_phase_hackathon_consensus_PWM_JABBAR_20260927/ /Subsystem/Subsystem1/Hardware M4/Power losses branch 2 ==
  note: Output signals
  note: Input signals
  note: Power losses calculations
  note: Note:
      | Power losses are modelled but not used in this specific simulation since they are small for a MMC module (low switching frequency).
      |
      | This power losses estimation can't be used when High voltage is 0.
  VHigh : Inport
  ILow : Inport  Port=2
  VLow : Inport  Port=3
  Add : Sum  Commented=on  Inputs=++++
  Branch DT loss : MATLAB Function  Commented=on  TreatAsAtomicUnit=on
  Branch cond loss : MATLAB Function  Commented=on  TreatAsAtomicUnit=on
  Branch gate loss : MATLAB Function  Commented=on  TreatAsAtomicUnit=on
  Branch switching loss : MATLAB Function  Commented=on  TreatAsAtomicUnit=on
  Divide1 : Product  Commented=on  Inputs=/*
  From : From  Commented=on  GotoTag=VHigh
  From1 : From  Commented=on  GotoTag=VLow
  From2 : From  Commented=on  GotoTag=ILow
  Goto3 : Goto  Commented=on  GotoTag=ILoss
  i1Loss : Outport
  wires:
  Branch switching loss/1(twist_FET_Psw) -> Add/2
  From2/1 -> Branch switching loss/2(ILow), Branch cond loss/3(ILow), Branch DT loss/1(ILow)
  Branch gate loss/1(twist_FET_Pg) -> Add/1
  Branch cond loss/1(twist_FET_Pcond) -> Add/4
  From/1 -> Divide1/1, Branch cond loss/1(VHigh), Branch switching loss/1(VHigh)
  Branch DT loss/1(twist_FET_Pdt) -> Add/3
  From1/1 -> Branch cond loss/2(VLow)
  Divide1/1 -> Goto3/1  "i1Loss"
  VHigh/1 -> [VHigh]
  ILow/1 -> [ILow]
  VLow/1 -> [VLow]
  [ILoss] -> i1Loss/1
  Add/1 -> Divide1/2

== system MMC_phase_hackathon_consensus_PWM_JABBAR_20260927/ /Subsystem/Subsystem1/Hardware M5/Driver block 1 ==
  command_Q1 : Inport
  command_Q2 : Inport  Port=2
  Q1 : Outport
  Q2 : Outport  Port=2
  wires:
  command_Q1/1 -> Q1/1
  command_Q2/1 -> Q2/1

== system MMC_phase_hackathon_consensus_PWM_JABBAR_20260927/ /Subsystem/Subsystem1/Hardware M5/Driver block 2 ==
  command_Q3 : Inport
  command_Q4 : Inport  Port=2
  Q3 : Outport
  Q4 : Outport  Port=2
  wires:
  command_Q3/1 -> Q3/1
  command_Q4/1 -> Q4/1

== system MMC_phase_hackathon_consensus_PWM_JABBAR_20260927/ /Subsystem/Subsystem1/Hardware M5/Feeder block ==
  note: Note:
      | Feeder chracteristics changed to consider threshold voltages (Vth_start = 9.7 V and Vth_stop = 8.9 V).
      | -When started, its VIN PIN consums the current generated by the lookup table fed with consumption experimental data from OwnTech.
      | -When stopped, its VIN PIN no longer consums current but its VCC PIN is modelled as a resistance calculated to match experimental results.
      | -When externally supply the 6 V used by the board, the feeder consums a constant 11.2 mA current when above threshold voltage, which is its correspondent to the minimum current in datasheet (15 mA).
  duty_cycle : Inport
  vHMeas : Inport  Port=2
  2-D Lookup Table : Lookup_n-D  Commented=on  LookupTableObject=feeder_current_tab  BreakpointsSpecification=Even spacing  BreakpointsForDimension1=[1:4]  BreakpointsForDimension2=[1:3]  BreakpointsForDimension1FirstPoint=feeder_VHigh_min  BreakpointsForDimension2FirstPoint=feeder_duty_min  BreakpointsForDimension1Spacing=feeder_VHigh_spacing  BreakpointsForDimension2Spacing=feeder_duty_spacing  TableSource=Input port  Table=feeder_current  InternalRulePriority=Speed  RndMeth=Simplest
      settings: InputPortMap=u0,u1,p221
  Constant11 : Constant  Commented=on  Value=is6VExternallySupplied
  Constant12 : Constant  Commented=on  Value=isFeederJumperOpen
  Constant2 : Constant  Commented=on  Value=0
  Constant4 : Constant  Commented=on  Value=0
  Constant5 : Constant  Commented=on
  Constant6 : Constant  Commented=on  Value=0
  Constant7 : Constant  Commented=on  Value=feeder_current_tab
  GreaterThan : RelationalOperator  Commented=on  Operator=>  OutDataTypeStr=boolean  RndMeth=Simplest  InputSameDT=off
  MATLAB Function : MATLAB Function  Commented=on  TreatAsAtomicUnit=on
  Memory : Memory  Commented=on  InheritSampleTime=on  LinearizeAsDelay=on
  Rate Limiter : RateLimiter  Commented=on  RisingSlewLimit=feeder_current_upper_rate_limit  FallingSlewLimit=feeder_current_lower_rate_limit  SampleTimeMode=inherited
  Switch : Switch  Commented=on  Criteria=u2 > Threshold  Threshold=2.05  SaturateOnIntegerOverflow=off  InputSameDT=off
  Switch10 : Switch  Commented=on  Criteria=u2 > Threshold  SaturateOnIntegerOverflow=off  InputSameDT=off
  Switch11 : Switch  Commented=on  Criteria=u2 > Threshold  SaturateOnIntegerOverflow=off  InputSameDT=off
  Switch9 : Switch  Commented=on  Criteria=u2 > Threshold  SaturateOnIntegerOverflow=off  InputSameDT=off
  Qjumper : Outport
  feeder_current : Outport  Port=2
  QVCC : Outport  Port=3
  wires:
  GreaterThan/1 -> Memory/1
  Constant2/1 -> GreaterThan/2
  Constant5/1 -> Switch11/3
  MATLAB Function/1(y) -> GreaterThan/1, Rate Limiter/1
  Constant4/1 -> Switch/3
  Switch/1 -> QVCC/1
  Switch10/1 -> Switch/1
  Memory/1 -> MATLAB Function/4(active_1)
  Constant6/1 -> Switch11/1, Switch10/1, Switch9/1
  Constant12/1 -> Switch11/2, Switch9/2, Switch10/2
  Constant11/1 -> MATLAB Function/3(isfeederdisabled)
  2-D Lookup Table/1 -> MATLAB Function/1(i_feeder)
  Rate Limiter/1 -> Switch9/3
  MATLAB Function/2(Q_VCC) -> Switch10/3
  Switch9/1 -> feeder_current/1
  Constant7/1 -> 2-D Lookup Table/3
  duty_cycle/1 -> 2-D Lookup Table/2
  vHMeas/1 -> MATLAB Function/2(vC), Switch/2, 2-D Lookup Table/1
  Switch11/1 -> Qjumper/1

== system MMC_phase_hackathon_consensus_PWM_JABBAR_20260927/ /Subsystem/Subsystem1/Hardware M5/HRTimA_1 ==
  note: PWM Timer Model
  note: Note 2:
      | All sampling times inferior than Ts = 1e-6 were desactivated or changed to Ts to reduce simulation duration
  note: Note 3:
      | PWM generator original resolution value at 100 ns
  note: Note 1:
      | HRTim modified adding block mode, equivalent to shield.power.stop(ALL);
  Duty cycle input : Inport
  Block : Inport  Port=2
  Constant : Constant  Value=0
  Dead Time : TransportDelay  Commented=on  DelayTime=twist_dead_time
  Demux : Demux  Outputs=2
  Logical Operator : Logic  AllPortsSameDT=off  OutDataTypeStr=boolean
  PWM Generator (2-Level) : Subsystem  AncestorBlock=|  DialogController=POWERSYS.PowerSysDialog  LoadFcn=sps_rtmsupport('LoadFcn', gcbh);  StartFcn=sps_rtmsupport('StartFcn', gcbh);  StopFcn=sps_rtmsupport('StopFcn', gcbh);  BlockChoice=InternalUref  mask(PWM Generator (2-Level)){ModulatorType=Single-phase half-bridge (2 pulses), ModulatorMode=Unsynchronized, Fc=twist_freq_switching, Pc=288, nF=27, MinMax=[0 1], SamplingTechnique=Symmetrical regular (single edge), ModulatingSignals=off, m=0.8, Freq=60, Phase=0, Ts=Ts, ShowCarrierOutport=off}
      | spsPWMGenerator2LevelLib/PWM Generator
      | (2-Level)
      mask prompts: ModulatorType "Generator type:"; ModulatorMode "Mode of operation:"; Fc "Frequency (Hz):"; Pc "Initial phase (degrees):"; nF "Switching ratio (carrier frequency / output frequency):"; MinMax "Minimum and maximum values: [ Min  Max ]"; SamplingTechnique "Sampling technique:"; ModulatingSignals "Internal generation of reference signal"; m "Modulation index:"; Freq "Frequency (Hz):"; Phase "Phase (degrees):"; Ts "Sample time (s):"; ShowCarrierOutport "Show measurement port"
      mask help:
      | Generate pulses for PWM-controlled 2-Level converter, using carrier-based two-level PWM method. The block can control switching devices of single-phase half-bridge, single-phase full-bridge (unipolar or bipolar modulation) or three-phase bridge.
      |
      | When the Synchronized mode of operation is selected, a second input is added to the block, and the internal generation of modulating signal is disabled. Use input 2 (wt) to synchronize the carrier.
      mask init:
      | sps = powericon('PWMGenerator2LevelInit',gcb,ModulatorType,SamplingTechnique,ModulatorMode,nF,Fc,MinMax,Pc,ShowCarrierOutport,ModulatingSignals,m,Freq,Phase,Ts);
      settings: CopyFcn=sps_rtmsupport('CopyFcn', gcbh);  DeleteFcn=sps_rtmsupport('DeleteFcn', gcbh);  UndoDeleteFcn=sps_rtmsupport('UndoDeleteFcn', gcbh);  ModelCloseFcn=sps_rtmsupport('ModelCloseFcn', gcbh);  PreSaveFcn=sps_rtmsupport('PreSaveFcn', gcbh);  PostSaveFcn=sps_rtmsupport('PostSaveFcn', gcbh);  NameChangeFcn=sps_rtmsupport('NameChangeFcn', gcbh);  PreCopyFcn=sps_rtmsupport('PreCopyFcn', gcbh);  OpenFcn="sps_rtmsupport('OpenFcn', gcbh, [1   2   7   8  13]);"  CloseFcn=sps_rtmsupport('CloseFcn', gcbh);  PreDeleteFcn=sps_rtmsupport('PreDeleteFcn', gcbh);
      mask Help: helpview(psbhelp);
      mask TypeOptions ModulatorType: Single-phase half-bridge (2 pulses) | Single-phase full-bridge (4 pulses) | Single-phase full-bridge - Bipolar modulation (4 pulses) | Three-phase bridge (6 pulses)
      mask TypeOptions ModulatorMode: Synchronized | Unsynchronized
      mask Callback ModulatorMode: powericon('PWMGenerator2LevelCback',gcb);
      mask TypeOptions SamplingTechnique: Natural | Asymmetrical regular (double edge) | Symmetrical regular (single edge)
      mask Callback ModulatingSignals: powericon('PWMGenerator2LevelCback',gcb);
      mask DialogControl Container3 Prompt: Carrier
      mask DialogControl ModulatingSignalParameters Prompt: Reference signal
  Peak acq : ZeroOrderHold  Commented=on  SampleTime=twist_data_acquisition_delay
  Switch : Switch  Criteria=u2 > Threshold  SaturateOnIntegerOverflow=off  InputSameDT=off
  Switch1 : Switch  Criteria=u2 > Threshold  SaturateOnIntegerOverflow=off  InputSameDT=off
  High-Side Q : Outport
  Low-Side Q : Outport  Port=2
  Carry Leg : Outport  Port=3
  wires:
  Demux/1 -> Switch/3  "high side"
  Duty cycle input/1 -> PWM Generator (2-Level)/1(Uref)  "duty_cycle"
  PWM Generator (2-Level)/2(Carry) -> Carry Leg/1, Peak acq/1  "carrier"
  Block/1 -> Switch/2, Switch1/2  "block"
  Demux/2 -> Switch1/3  "low side"
  Switch1/1 -> Low-Side Q/1
  Switch/1 -> High-Side Q/1
  Constant/1 -> Switch1/1, Switch/1
  PWM Generator (2-Level)/1(P) -> Demux/1, Dead Time/1, Logical Operator/1, Logical Operator/2  "PWM_out"
